simulink model "IL_oswec_hydraulic"  (R2025b)
settings: Solver=ode45  StartTime=0  StopTime=300  FixedStep=0.1  MaxStep=0.1  RelTol=1e-3  AbsTol=1e-3
libraries: SimscapeFluids_lib x12, fl_lib x12, nesl_utility x4, customization_lib x1
settings Model: Creator=ndegoede  LastModifiedBy=ndegoede
settings SolverCC: AutoScaleAbsTol=off  DaesscMode=FullDebug  ZeroCrossControl=DisableAll  AutoInsertRateTranBlk=on  DecoupledContinuousIntegration=on
settings DataIOCC: ReturnWorkspaceOutputs=off
settings OptimizationCC: SimCompilerOptimization=on
settings SimscapeCC: SimscapeLogType=all  SimscapeLogOpenViewer=on

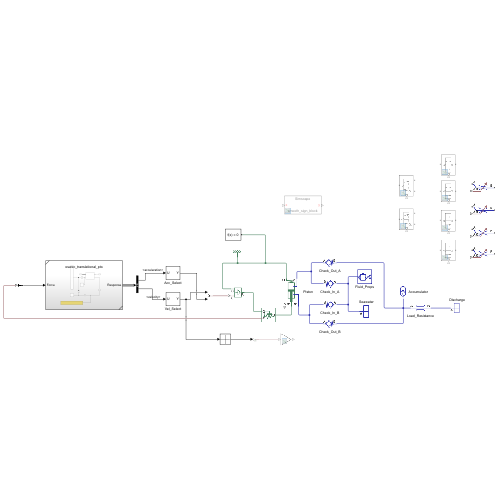
[thumbnail: Simulink's stored preview of the top-level diagram]
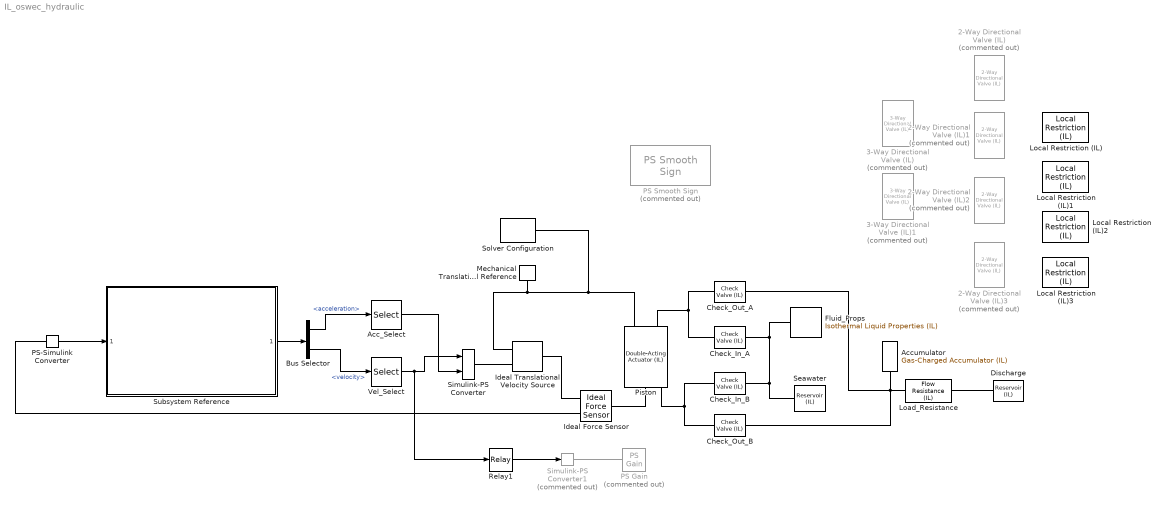
== system IL_oswec_hydraulic ==
  2-Way Directional Valve (IL){,1..3} (4 alike) : SimscapeFluids_lib/Isothermal Liquid/Valves & Orifices/Directional Control Valves/2-Way Directional Valve (IL)  Commented=on  valve_spec=fluids.isothermal_liquid.valves_orifices.directional_control_valves.enum.directional_valve_spec.linear  S_max=1 m  del_S_max=1 m  area_max=0.05 m^2  area_leak=1e-8 m^2  del_S_TLU=[0, .002, .004, .007, .017] m  orifice_area_TLU=[1e-09, 2.0352e-07, 4.0736e-05, .00011438, .00034356] m^2  del_S_vol_flow_TLU=[0, .002, .004, .007, .017] m  p_diff_TLU=[.3, .5, .7] MPa  vol_flow_TLU=1e-3 * [1.7e-05, 2e-05, 2.6e-05; .0035, .0045, .0053; .7, .9, 1.06; 1.96, 2.5, 3; 6, 7.7, 9.13] m^3/s  Cd=0.7  Re_c=150  smoothing_factor=0  pressure_recovery=false  area=inf m^2
      settings: InternalSimscapePortConfiguration="{\"Bottom\":[{\"id\":\"B\",\"label\":\"B\",\"type\":\"foundation.isothermal_liquid.isothermal_liquid\"}],\"Left\":[{\"id\":\"S\",\"label\":\"S\",\"type\":\"input\"}],\"Right\":[],\"Top\":[{\"id\":\"A\",\"label\":\"A\",\"type\":\"foundation.isothermal_liquid.isothermal_liquid\"}]}"
  3-Way Directional Valve (IL) : SimscapeFluids_lib/Isothermal Liquid/Valves & Orifices/Directional Control Valves/3-Way Directional Valve (IL)  Commented=on  open_orifices_pos=fluids.isothermal_liquid.valves_orifices.directional_control_valves.enum.DirectionalValveOpenOrifices3Way.PA  open_orifices_neg=fluids.isothermal_liquid.valves_orifices.directional_control_valves.enum.DirectionalValveOpenOrifices3Way.AT  area_spec=fluids.isothermal_liquid.valves_orifices.directional_control_valves.enum.directional_valve_area_spec.identical  valve_spec=fluids.isothermal_liquid.valves_orifices.directional_control_valves.enum.directional_valve_spec.linear  del_S_max=1 m  area_max=0.05 m^2  del_S_TLU=[0, .00125, .0025, .00375, .005] m  valve_area_TLU=[1e-10, 1e-05, 4e-05, 8e-05, .0001] m^2  del_S_vol_flow_TLU=[0, .00125, .0025, .00375, .005] m  p_diff_TLU=[-.1, .3, .5, .7] MPa  vol_flow_TLU=[-9.05e-10, 1.57e-09, 2.02e-09, 2.39e-09; -9.05e-05, .000157, .000202, .000239; -.000362, .000627, .00081, .000958; -.000724, .00125, .00162, .00192; -.000905, .00156, .002, .00239] m^3/s  area=inf m^2  area_leak=1e-10 m^2  Cd=0.7  Re_c=150  smoothing_factor=0.01  pressure_recovery=false  S_max_PA=4.5e-3 m  del_S_max_PA=0.005 m  area_max_PA=1e-4 m^2  del_S_TLU_PA=[0, .00125, .0025, .00375, .005] m  valve_area_TLU_PA=[1e-10, 1e-05, 4e-05, 8e-05, .0001] m^2  del_S_vol_flow_TLU_PA=[0, .00125, .0025, .00375, .005] m  p_diff_TLU_PA=[-.1, .3, .5, .7] MPa  vol_flow_TLU_PA=[-9.05e-10, 1.57e-09, 2.02e-09, 2.39e-09; -9.05e-05, .000157, .000202, .000239; -.000362, .000627, .00081, .000958; -.000724, .00125, .00162, .00192; -.000905, .00156, .002, .00239] m^3/s  S_max_AT=-4.5e-3 m  del_S_max_AT=0.005 m  area_max_AT=1e-4 m^2  del_S_TLU_AT=[0, .00125, .0025, .00375, .005] m  valve_area_TLU_AT=[1e-10, 1e-05, 4e-05, 8e-05, .0001] m^2  del_S_vol_flow_TLU_AT=[0, .00125, .0025, .00375, .005] m  p_diff_TLU_AT=[-.1, .3, .5, .7] MPa  vol_flow_TLU_AT=[-9.05e-10, 1.57e-09, 2.02e-09, 2.39e-09; -9.05e-05, .000157, .000202, .000239; -.000362, .000627, .00081, .000958; -.000724, .00125, .00162, .00192; -.000905, .00156, .002, .00239] m^3/s  S_max_PT=4.5e-3 m  del_S_max_PT=0.005 m  area_max_PT=1e-4 m^2  del_S_TLU_PT=[0, .00125, .0025, .00375, .005] m  valve_area_TLU_PT=[1e-10, 1e-05, 4e-05, 8e-05, .0001] m^2  del_S_vol_flow_TLU_PT=[0, .00125, .0025, .00375, .005] m  p_diff_TLU_PT=[-.1, .3, .5, .7] MPa  vol_flow_TLU_PT=[-9.05e-10, 1.57e-09, 2.02e-09, 2.39e-09; -9.05e-05, .000157, .000202, .000239; -.000362, .000627, .00081, .000958; -.000724, .00125, .00162, .00192; -.000905, .00156, .002, .00239] m^3/s
      settings: InternalSimscapePortConfiguration="{\"Bottom\":[{\"id\":\"P\",\"label\":\"P\",\"type\":\"foundation.isothermal_liquid.isothermal_liquid\"},{\"id\":\"T\",\"label\":\"T\",\"type\":\"foundation.isothermal_liquid.isothermal_liquid\"}],\"Left\":[{\"id\":\"S\",\"label\":\"S\",\"type\":\"input\"}],\"Right\":[],\"Top\":[{\"id\":\"A\",\"label\":\"A\",\"type\":\"foundation.isothermal_liquid.isothermal_liquid\"}]}"
  3-Way Directional Valve (IL)1 : SimscapeFluids_lib/Isothermal Liquid/Valves & Orifices/Directional Control Valves/3-Way Directional Valve (IL)  Commented=on  open_orifices_pos=fluids.isothermal_liquid.valves_orifices.directional_control_valves.enum.DirectionalValveOpenOrifices3Way.PA  open_orifices_neg=fluids.isothermal_liquid.valves_orifices.directional_control_valves.enum.DirectionalValveOpenOrifices3Way.AT  area_spec=fluids.isothermal_liquid.valves_orifices.directional_control_valves.enum.directional_valve_area_spec.identical  valve_spec=fluids.isothermal_liquid.valves_orifices.directional_control_valves.enum.directional_valve_spec.linear  del_S_max=1 m  area_max=0.05 m^2  del_S_TLU=[0, .00125, .0025, .00375, .005] m  valve_area_TLU=[1e-10, 1e-05, 4e-05, 8e-05, .0001] m^2  del_S_vol_flow_TLU=[0, .00125, .0025, .00375, .005] m  p_diff_TLU=[-.1, .3, .5, .7] MPa  vol_flow_TLU=[-9.05e-10, 1.57e-09, 2.02e-09, 2.39e-09; -9.05e-05, .000157, .000202, .000239; -.000362, .000627, .00081, .000958; -.000724, .00125, .00162, .00192; -.000905, .00156, .002, .00239] m^3/s  area=inf m^2  area_leak=1e-10 m^2  Cd=0.7  Re_c=150  smoothing_factor=0.01  pressure_recovery=false  S_max_PA=4.5e-3 m  del_S_max_PA=0.005 m  area_max_PA=1e-4 m^2  del_S_TLU_PA=[0, .00125, .0025, .00375, .005] m  valve_area_TLU_PA=[1e-10, 1e-05, 4e-05, 8e-05, .0001] m^2  del_S_vol_flow_TLU_PA=[0, .00125, .0025, .00375, .005] m  p_diff_TLU_PA=[-.1, .3, .5, .7] MPa  vol_flow_TLU_PA=[-9.05e-10, 1.57e-09, 2.02e-09, 2.39e-09; -9.05e-05, .000157, .000202, .000239; -.000362, .000627, .00081, .000958; -.000724, .00125, .00162, .00192; -.000905, .00156, .002, .00239] m^3/s  S_max_AT=-4.5e-3 m  del_S_max_AT=0.005 m  area_max_AT=1e-4 m^2  del_S_TLU_AT=[0, .00125, .0025, .00375, .005] m  valve_area_TLU_AT=[1e-10, 1e-05, 4e-05, 8e-05, .0001] m^2  del_S_vol_flow_TLU_AT=[0, .00125, .0025, .00375, .005] m  p_diff_TLU_AT=[-.1, .3, .5, .7] MPa  vol_flow_TLU_AT=[-9.05e-10, 1.57e-09, 2.02e-09, 2.39e-09; -9.05e-05, .000157, .000202, .000239; -.000362, .000627, .00081, .000958; -.000724, .00125, .00162, .00192; -.000905, .00156, .002, .00239] m^3/s  S_max_PT=4.5e-3 m  del_S_max_PT=0.005 m  area_max_PT=1e-4 m^2  del_S_TLU_PT=[0, .00125, .0025, .00375, .005] m  valve_area_TLU_PT=[1e-10, 1e-05, 4e-05, 8e-05, .0001] m^2  del_S_vol_flow_TLU_PT=[0, .00125, .0025, .00375, .005] m  p_diff_TLU_PT=[-.1, .3, .5, .7] MPa  vol_flow_TLU_PT=[-9.05e-10, 1.57e-09, 2.02e-09, 2.39e-09; -9.05e-05, .000157, .000202, .000239; -.000362, .000627, .00081, .000958; -.000724, .00125, .00162, .00192; -.000905, .00156, .002, .00239] m^3/s
      settings: InternalSimscapePortConfiguration="{\"Bottom\":[{\"id\":\"P\",\"label\":\"P\",\"type\":\"foundation.isothermal_liquid.isothermal_liquid\"},{\"id\":\"T\",\"label\":\"T\",\"type\":\"foundation.isothermal_liquid.isothermal_liquid\"}],\"Left\":[{\"id\":\"S\",\"label\":\"S\",\"type\":\"input\"}],\"Right\":[],\"Top\":[{\"id\":\"A\",\"label\":\"A\",\"type\":\"foundation.isothermal_liquid.isothermal_liquid\"}]}"
  Acc_Select : Selector  InputPortWidth=6  IndexOptions=Index vector (dialog)  Indices=3  OutputSizes=1
  Accumulator : SimscapeFluids_lib/Isothermal Liquid/Tanks & Accumulators/Gas-Charged Accumulator (IL)  capacity=4 m^3  dead_volume=4e-5 m^3  p_precharge=3 MPa  k_sh=1.4  stiff_coeff=1e4 MPa/m^3  dynamic_compressibility=true  liquid_volume_specify=off  liquid_volume_priority=High  liquid_volume=5e-3 m^3  liquid_volume_nominal_specify=off  liquid_volume_nominal_value=1  liquid_volume_nominal_unit=m^3  liquid_mass_specify=off  liquid_mass_priority=None  liquid_mass=5 kg  liquid_mass_nominal_specify=off  liquid_mass_nominal_value=1  liquid_mass_nominal_unit=kg  p_I_specify=off  p_I_priority=None  p_I=0.101325 MPa  p_I_nominal_specify=off  p_I_nominal_value=1  p_I_nominal_unit=MPa
      settings: InternalSimscapePortConfiguration="{\"Bottom\":[],\"Left\":[],\"Right\":[{\"id\":\"A\",\"label\":\"A\",\"type\":\"foundation.isothermal_liquid.isothermal_liquid\"}],\"Top\":[]}"
  Bus Selector : BusSelector  OutputSignals=acceleration,velocity
  Check_In_A : SimscapeFluids_lib/Isothermal Liquid/Valves & Orifices/Directional Control Valves/Check Valve (IL)  opening_spec=fluids.isothermal_liquid.valves_orifices.enum.PressureOpeningSpec.Linear  pressure_control_spec=fluids.isothermal_liquid.valves_orifices.enum.pressure_control_spec.dp  p_crack_differential=0.01 MPa  p_crack_gauge=0.1 MPa  press_max_differential=0.1 MPa  press_max_gauge=0.2 MPa  area_max=0.05 m^2  area_leak=1e-8 m^2  p_diff_TLU=[0.01 : 0.01 : 0.1] MPa  valve_area_TLU=[1e-10, 1e-05, 2e-05, 3e-05, 4e-05, 5e-05, 6e-05, 7.5e-05, 8.5e-05, .0001] m^2  vol_flow_TLU=[.000358, .045, .11, .191, .284, .39, .505, .63, .764, .905] .* 1e-3 m^3/s  area=inf m^2  Cd=0.7  Re_c=150  smoothing_factor=0.01  pressure_recovery=false  opening_dynamics=false  tau=0.1 s
      settings: InternalSimscapePortConfiguration="{\"Bottom\":[],\"Left\":[{\"id\":\"A\",\"label\":\"A\",\"type\":\"foundation.isothermal_liquid.isothermal_liquid\"}],\"Right\":[{\"id\":\"B\",\"label\":\"B\",\"type\":\"foundation.isothermal_liquid.isothermal_liquid\"}],\"Top\":[]}"
  Check_In_B : SimscapeFluids_lib/Isothermal Liquid/Valves & Orifices/Directional Control Valves/Check Valve (IL)  opening_spec=fluids.isothermal_liquid.valves_orifices.enum.PressureOpeningSpec.Linear  pressure_control_spec=fluids.isothermal_liquid.valves_orifices.enum.pressure_control_spec.dp  p_crack_differential=0.01 MPa  p_crack_gauge=0.1 MPa  press_max_differential=0.1 MPa  press_max_gauge=0.2 MPa  area_max=0.05 m^2  area_leak=1e-8 m^2  p_diff_TLU=[0.01 : 0.01 : 0.1] MPa  valve_area_TLU=[1e-10, 1e-05, 2e-05, 3e-05, 4e-05, 5e-05, 6e-05, 7.5e-05, 8.5e-05, .0001] m^2  vol_flow_TLU=[.000358, .045, .11, .191, .284, .39, .505, .63, .764, .905] .* 1e-3 m^3/s  area=inf m^2  Cd=0.7  Re_c=150  smoothing_factor=0.01  pressure_recovery=false  opening_dynamics=false  tau=0.1 s
      settings: InternalSimscapePortConfiguration="{\"Bottom\":[],\"Left\":[{\"id\":\"A\",\"label\":\"A\",\"type\":\"foundation.isothermal_liquid.isothermal_liquid\"}],\"Right\":[{\"id\":\"B\",\"label\":\"B\",\"type\":\"foundation.isothermal_liquid.isothermal_liquid\"}],\"Top\":[]}"
  Check_Out_A : SimscapeFluids_lib/Isothermal Liquid/Valves & Orifices/Directional Control Valves/Check Valve (IL)  opening_spec=fluids.isothermal_liquid.valves_orifices.enum.PressureOpeningSpec.Linear  pressure_control_spec=fluids.isothermal_liquid.valves_orifices.enum.pressure_control_spec.dp  p_crack_differential=0.01 MPa  p_crack_gauge=0.1 MPa  press_max_differential=0.1 MPa  press_max_gauge=0.2 MPa  area_max=0.05 m^2  area_leak=1e-8 m^2  p_diff_TLU=[0.01 : 0.01 : 0.1] MPa  valve_area_TLU=[1e-10, 1e-05, 2e-05, 3e-05, 4e-05, 5e-05, 6e-05, 7.5e-05, 8.5e-05, .0001] m^2  vol_flow_TLU=[.000358, .045, .11, .191, .284, .39, .505, .63, .764, .905] .* 1e-3 m^3/s  area=inf m^2  Cd=0.7  Re_c=150  smoothing_factor=0.01  pressure_recovery=false  opening_dynamics=false  tau=0.1 s
      settings: InternalSimscapePortConfiguration="{\"Bottom\":[],\"Left\":[{\"id\":\"A\",\"label\":\"A\",\"type\":\"foundation.isothermal_liquid.isothermal_liquid\"}],\"Right\":[{\"id\":\"B\",\"label\":\"B\",\"type\":\"foundation.isothermal_liquid.isothermal_liquid\"}],\"Top\":[]}"
  Check_Out_B : SimscapeFluids_lib/Isothermal Liquid/Valves & Orifices/Directional Control Valves/Check Valve (IL)  opening_spec=fluids.isothermal_liquid.valves_orifices.enum.PressureOpeningSpec.Linear  pressure_control_spec=fluids.isothermal_liquid.valves_orifices.enum.pressure_control_spec.dp  p_crack_differential=0.01 MPa  p_crack_gauge=0.1 MPa  press_max_differential=0.1 MPa  press_max_gauge=0.2 MPa  area_max=0.05 m^2  area_leak=1e-8 m^2  p_diff_TLU=[0.01 : 0.01 : 0.1] MPa  valve_area_TLU=[1e-10, 1e-05, 2e-05, 3e-05, 4e-05, 5e-05, 6e-05, 7.5e-05, 8.5e-05, .0001] m^2  vol_flow_TLU=[.000358, .045, .11, .191, .284, .39, .505, .63, .764, .905] .* 1e-3 m^3/s  area=inf m^2  Cd=0.7  Re_c=150  smoothing_factor=0.01  pressure_recovery=false  opening_dynamics=false  tau=0.1 s
      settings: InternalSimscapePortConfiguration="{\"Bottom\":[],\"Left\":[{\"id\":\"A\",\"label\":\"A\",\"type\":\"foundation.isothermal_liquid.isothermal_liquid\"}],\"Right\":[{\"id\":\"B\",\"label\":\"B\",\"type\":\"foundation.isothermal_liquid.isothermal_liquid\"}],\"Top\":[]}"
  Discharge : fl_lib/Isothermal Liquid/Elements/Reservoir (IL)  reservoir_type=foundation.enum.constant_controlled.constant  pressure_spec=foundation.enum.pressure_spec.specified  reservoir_pressure=3 MPa
  Fluid_Props : fl_lib/Isothermal Liquid/Utilities/Isothermal Liquid Properties (IL)  rho_L_atm=1025 kg/m^3  bulk_modulus_model=foundation.enum.bulk_modulus_model.const  beta_gain=6  beta_L_atm=2.1791e9 Pa  nu_atm=1.08e-6 m^2/s  p_atm=0.101325 MPa  p_min=1 Pa  properties_range_check=simscape.enum.assert.action.error  air_fraction=0.005  polytropic_index=1.0  rho_g_atm=1.225 kg/m^3  air_dissolution_model=false  p_crit=3 MPa
  Ideal Force Sensor : fl_lib/Mechanical/Mechanical Sensors/Ideal Force Sensor
  Ideal Translational Velocity Source : fl_lib/Mechanical/Mechanical Sources/Ideal Translational Velocity Source
  Load_Resistance : fl_lib/Isothermal Liquid/Elements/Flow Resistance (IL)  delta_p_nominal=0.0627/5 MPa  mdot_nominal=1 kg/s  laminar_fraction=1e-3
      settings: InternalSimscapePortConfiguration="{\"Bottom\":[],\"Left\":[{\"id\":\"A\",\"label\":\"A\",\"type\":\"foundation.isothermal_liquid.isothermal_liquid\"}],\"Right\":[{\"id\":\"B\",\"label\":\"B\",\"type\":\"foundation.isothermal_liquid.isothermal_liquid\"}],\"Top\":[]}"
  Local Restriction (IL){,1..3} (4 alike) : fl_lib/Isothermal Liquid/Elements/Local Restriction (IL)  restriction_type=foundation.enum.restriction_type.variable  restriction_area=1e-3 m^2  min_area=1e-8 m^2  max_area=0.05 m^2  area=inf m^2  Cd=0.7  Re_c=150  pressure_recovery=false
      settings: InternalSimscapePortConfiguration="{\"Bottom\":[],\"Left\":[{\"id\":\"A\",\"label\":\"A\",\"type\":\"foundation.isothermal_liquid.isothermal_liquid\"},{\"id\":\"AR\",\"label\":\"AR\",\"type\":\"input\"}],\"Right\":[{\"id\":\"B\",\"label\":\"B\",\"type\":\"foundation.isothermal_liquid.isothermal_liquid\"}],\"Top\":[]}"
  Mechanical Translational Reference : fl_lib/Mechanical/Translational Elements/Mechanical Translational Reference
  PS Gain : fl_lib/Physical Signals/Functions/PS Gain  Commented=on  gain=-1
  PS Smooth Sign : customization_lib/function/PS Smooth Sign  Commented=on  x_th=1e-12
      settings: SourceProductName=Customization  InternalSimscapePortConfiguration="{\"Bottom\":[],\"Left\":[{\"id\":\"x\",\"label\":\"x\",\"type\":\"input\"}],\"Right\":[{\"id\":\"y\",\"label\":\"y\",\"type\":\"output\"}],\"Top\":[]}"
  PS-Simulink Converter : nesl_utility/PS-Simulink Converter  PhysicalDomain=network_engine_domain  SubClassName=ps_output  LeftPortType=input  RightPortType=output  PseudoPeriodic=off  Frequencies=[]  VectorFormat=inherit  Unit=inherit  AffineConversion=off
  Piston : SimscapeFluids_lib/Isothermal Liquid/Actuators/Double-Acting Actuator (IL)  single_fluid=true  mech_orientation=foundation.enum.MechOrientationTranslational.Positive  piston_area_A=0.26 m^2  piston_area_B=0.26 m^2  stroke=14 m  dead_volume_A=2*0.26 m^3  dead_volume_B=2*0.26 m^3  pressure_spec=foundation.enum.pressure_spec.atmospheric  environment_pressure=0.101325 MPa  hardstop_model=simscape.enum.hardstop.smooth  stiff_coeff=1e10 N/m  damping_coeff=150 N*s/m  transition=0.1 mm  coeff_rest=0.7  v_tol=0.001 m/s  f_tol=0.001 N  cushion_A_spec=false  area_plunger_A=1e-4 m^2  length_plunger_A=1e-3 m  area_cushion_orifice_A=1e-6 m^2  area_leak_plunger_A=1e-7 m^2  p_crack_differential_A=0.01 MPa  press_max_differential_A=0.1 MPa  check_valve_area_max_A=0.05 m^2  check_valve_area_leak_A=1e-6 m^2  smoothing_factor_A=0.01  cushion_B_spec=false  area_plunger_B=1e-4 m^2  length_plunger_B=1e-3 m  area_cushion_orifice_B=1e-6 m^2  area_leak_plunger_B=1e-7 m^2  p_crack_differential_B=0.01 MPa  press_max_differential_B=0.1 MPa  check_valve_area_max_B=0.05 m^2  check_valve_area_leak_B=1e-6 m^2  smoothing_factor_B=0.01  friction_spec=false  breakaway_Coulomb_ratio=1.2  breakaway_velocity=0.1 m/s  preload_force=20 N  Coulomb_coeff=1e-6 N/Pa  viscous_coeff=100 N*s/m  leakage_spec=false  clearance=1e-4 m  piston_length=0.01 m  displacement_spec=foundation.enum.DisplacementSpec.Calculate  x0=7 m  dynamic_compressibility=false  p0_A=P_ocean MPa  p0_B=P_ocean MPa  p_nominal_A=0.101325 MPa  p_nominal_B=0.101325 MPa
      settings: InternalSimscapePortConfiguration="{\"Bottom\":[],\"Left\":[{\"id\":\"C\",\"label\":\"C\",\"type\":\"foundation.mechanical.translational.translational\"},{\"id\":\"A\",\"label\":\"A\",\"type\":\"foundation.isothermal_liquid.isothermal_liquid\"}],\"Right\":[{\"id\":\"p_out\",\"label\":\"p\",\"type\":\"output\"},{\"id\":\"R\",\"label\":\"R\",\"type\":\"foundation.mechanical.translational.translational\"},{\"id\":\"B\",\"label\":\"B\",\"type\":\"foundation.isothermal_liquid.isothermal_liquid\"}],\"Top\":[]}"
  Relay1 : Relay  OnSwitchValue=0  OffSwitchValue=0  OffOutputValue=-1
  Seawater : fl_lib/Isothermal Liquid/Elements/Reservoir (IL)  reservoir_type=foundation.enum.constant_controlled.constant  pressure_spec=foundation.enum.pressure_spec.specified  reservoir_pressure=P_ocean MPa
  Simulink-PS Converter : nesl_utility/Simulink-PS Converter  PhysicalDomain=network_engine_domain  SubClassName=ps_input  LeftPortType=input  RightPortType=output  PseudoPeriodic=off  Frequencies=[]  NoiseDistribution=none  NoiseParameters=[]  Unit=1  AffineConversion=off  FilteringAndDerivatives=provide  SimscapeFilterOrder=1  InputFilterTimeConstant=0.001  UdotUserProvided=1
  Simulink-PS Converter1 : nesl_utility/Simulink-PS Converter  Commented=on  PhysicalDomain=network_engine_domain  SubClassName=ps_input  LeftPortType=input  RightPortType=output  PseudoPeriodic=off  Frequencies=[]  NoiseDistribution=none  NoiseParameters=[]  Unit=1  AffineConversion=off  FilteringAndDerivatives=zero  SimscapeFilterOrder=1  InputFilterTimeConstant=0.001  UdotUserProvided=0
  Solver Configuration : nesl_utility/Solver Configuration  PhysicalDomain=network_engine_domain  SubClassName=solver  LeftPortType=input  RightPortType=generic  Tones=[]  Harmonics=[]  SimulateNoise=off  Profile=off  UseLocalSampling=off  EnableSwitchedLinearOptims=on  FrequencyDomain=off  UseCCode=off  RelTol=0.001  AbsTol=0.001  MinStep=1e-09  ToWorkspace=off  RevertToSquareIcSolve=off  NumHomotopyIterations=100  PhasorMode=off  PhasorModeNumHarmonics=1  ConsistencySolver=NEWTON_XTOL_AFTER_FTOL  IndexReductionMethod=DerivativeReplacement  DoDC=on  ResidualTolerance=1e-4  ConsistencyTolSource=GLOBAL  ConsistencyAbsTol=0.001  ConsistencyRelTol=0.001  ConsistencyTolFactor=0.001  UseLocalSolver=off  LocalSolverChoice=NE_BACKWARD_EULER_ADVANCER  ResolveIndetEquations=on  FunctionEvalNumThread=1  LocalSolverSampleTime=0.01  DoFixedCost=off  MaxNonlinIter=3  MaxModeIter=2  ComputeImpulses=off  ImpulseIterations=2  LinearAlgebra=auto  LinearAlgebraNumThread=0  EquationFormulation=NE_TIME_EF  DelaysMemoryBudget=1024  AutomaticFiltering=on  FilteringTimeConstant=0.001  PartitionStorageMethod=AS_NEEDED  PartitionMemoryBudget=1024  PartitionMethod=ROBUST  MultibodyUseLocalSolver=off  MultibodyLocalSolverChoice=ODE1  MultibodyLocalSolverSampleTime=0.001
  Subsystem Reference : Subsystem  ReferencedSubsystem=oswec_translational_pto
  Vel_Select : Selector  InputPortWidth=6  IndexOptions=Index vector (dialog)  Indices=3  OutputSizes=1
  wires:
  Subsystem Reference/1 -> Bus Selector/1
  Bus Selector/2 -> Vel_Select/1  "<velocity>"
  Vel_Select/1 -> Relay1/1, Simulink-PS Converter/1
  Bus Selector/1 -> Acc_Select/1  "<acceleration>"
  Acc_Select/1 -> Simulink-PS Converter/2
  PS-Simulink Converter/1 -> Subsystem Reference/1
  Relay1/1 -> Simulink-PS Converter1/1
  connections:
  Ideal Translational Velocity Source/RConn1 -- Simulink-PS Converter/RConn1
  Piston/LConn1 -- Mechanical Translational Reference/LConn1 -- Ideal Translational Velocity Source/RConn2 -- Solver Configuration/RConn1
  Fluid_Props/RConn1 -- Check_In_A/LConn1 -- Check_In_B/LConn1 -- Seawater/LConn1
  Load_Resistance/LConn1 -- Check_Out_B/RConn1 -- Check_Out_A/RConn1 -- Accumulator/RConn1
  Load_Resistance/RConn1 -- Discharge/LConn1
  Simulink-PS Converter1/RConn1 -- PS Gain/LConn1
  Ideal Translational Velocity Source/LConn1 -- Ideal Force Sensor/RConn1
  Ideal Force Sensor/LConn1 -- Piston/RConn2
  Ideal Force Sensor/RConn2 -- PS-Simulink Converter/LConn1
  Piston/RConn3 -- Check_In_B/RConn1 -- Check_Out_B/LConn1
  Piston/LConn2 -- Check_In_A/RConn1 -- Check_Out_A/LConn1
